simulink model "Gen3_J2_PMSM_Actuator"  (R2026b)
settings: Solver=ode23t  StopTime=1  MaxStep=1e-4  RelTol=1e-6  AbsTol=1e-8
model workspace (MAT data in the model file):
  p.Rs = 0.013
  p.Ld = 0.00019
  p.Lq = 0.00025
  p.pp = 6
  p.psi = 0.03
  p.Kt = 0.27
  p.N = 2
  p.Jtotal_motor = 0.0125
  p.Jm = 0.01
  p.Jload_test = 0.01
  p.Bm = 0
  p.Kpd = 0.19
  p.Kpq = 0.25
  p.Kid = 13
  p.Kiq = 13
  p.Imax = 1
  p.Vqmax = 1
  p.s = 1
  p.Kaw = 52
settings Model: Creator=rninh  LastModifiedBy=rninh

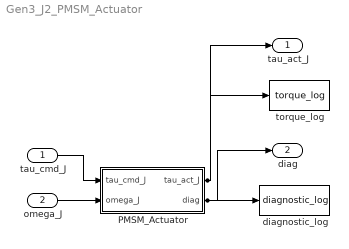
== system Gen3_J2_PMSM_Actuator ==
  tau_cmd_J : Inport  Unit=N*m  PortDimensions=1  Interpolate=off
  omega_J : Inport  Port=2  Unit=rad/s  PortDimensions=1  Interpolate=off
  PMSM_Actuator : Subsystem
  diagnostic_log : ToWorkspace  VariableName=diagnostic_log  SaveFormat=Timeseries  SampleTime=-1
  torque_log : ToWorkspace  VariableName=torque_log  SaveFormat=Timeseries  SampleTime=-1
  tau_act_J : Outport  Unit=N*m
  diag : Outport  Port=2
  wires:
  tau_cmd_J/1 -> PMSM_Actuator/1(tau_cmd_J)
  omega_J/1 -> PMSM_Actuator/2(omega_J)
  PMSM_Actuator/1(tau_act_J) -> tau_act_J/1, torque_log/1
  PMSM_Actuator/2(diag) -> diag/1, diagnostic_log/1

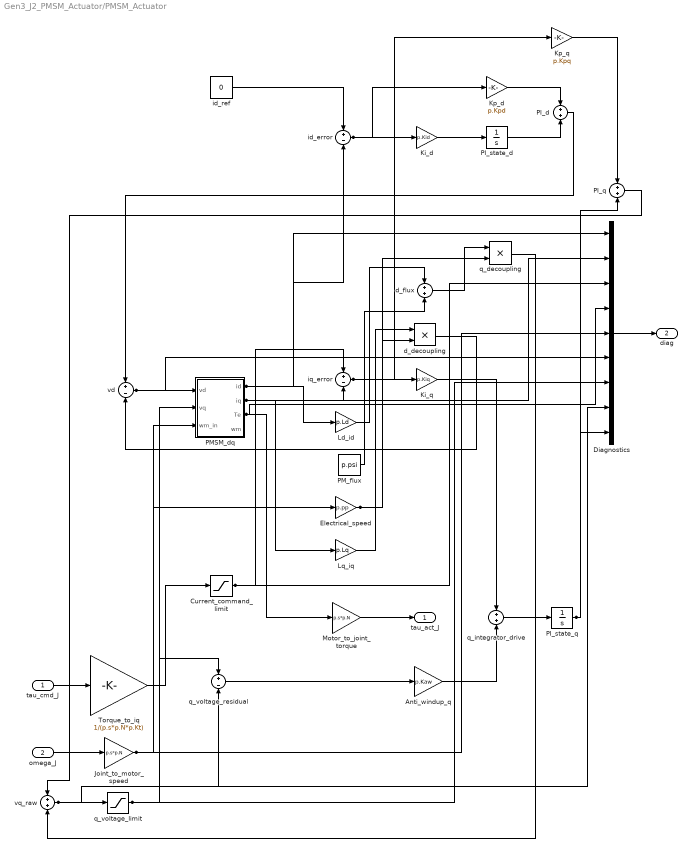
== system Gen3_J2_PMSM_Actuator/PMSM_Actuator ==
  tau_cmd_J : Inport  Unit=N*m  PortDimensions=1
  omega_J : Inport  Port=2  Unit=rad/s  PortDimensions=1
  Anti_windup_q : Gain  Gain=p.Kaw
  Current_command_limit : Saturate  UpperLimit=p.Imax  LowerLimit=-p.Imax
  Diagnostics : Mux  Inputs=9
  Electrical_speed : Gain  Gain=p.pp
  Joint_to_motor_speed : Gain  Gain=p.s*p.N
  Ki_d : Gain  Gain=p.Kid
  Ki_q : Gain  Gain=p.Kiq
  Kp_d : Gain  Gain=p.Kpd
  Kp_q : Gain  Gain=p.Kpq
  Ld_id : Gain  Gain=p.Ld
  Lq_iq : Gain  Gain=p.Lq
  Motor_to_joint_torque : Gain  Gain=p.s*p.N
  PI_d : Sum
  PI_q : Sum
  PI_state_d : Integrator
  PI_state_q : Integrator
  PMSM_dq : Subsystem
  PM_flux : Constant  Value=p.psi
  Torque_to_iq : Gain  Gain=1/(p.s*p.N*p.Kt)
  d_decoupling : Product
  d_flux : Sum
  id_error : Sum  Inputs=+-
  id_ref : Constant  Value=0
  iq_error : Sum  Inputs=+-
  q_decoupling : Product
  q_integrator_drive : Sum
  q_voltage_limit : Saturate  UpperLimit=p.Vqmax  LowerLimit=-p.Vqmax
  q_voltage_residual : Sum  Inputs=+-
  vd : Sum  Inputs=+-
  vq_raw : Sum
  tau_act_J : Outport  Unit=N*m  PortDimensions=1
  diag : Outport  Port=2
  wires:
  Joint_to_motor_speed/1 -> Electrical_speed/1, Diagnostics/5, PMSM_dq/3(wm_in)
  vd/1 -> Diagnostics/6, PMSM_dq/1(vd)
  PI_state_q/1 -> PI_q/2, Diagnostics/9
  tau_cmd_J/1 -> Torque_to_iq/1
  omega_J/1 -> Joint_to_motor_speed/1
  vq_raw/1 -> Diagnostics/8, q_voltage_residual/2, q_voltage_limit/1
  id_ref/1 -> id_error/1
  q_voltage_limit/1 -> q_voltage_residual/1, PMSM_dq/2(vq), Diagnostics/7
  Torque_to_iq/1 -> Current_command_limit/1
  d_flux/1 -> q_decoupling/1
  PMSM_dq/1(id) -> Diagnostics/1, id_error/2, Ld_id/1
  PMSM_dq/3(Te) -> Diagnostics/4, Motor_to_joint_torque/1
  PMSM_dq/2(iq) -> iq_error/2, Diagnostics/2, Lq_iq/1
  Current_command_limit/1 -> iq_error/1, Diagnostics/3
  q_voltage_residual/1 -> Anti_windup_q/1
  id_error/1 -> Kp_d/1, Ki_d/1
  iq_error/1 -> Kp_q/1, Ki_q/1
  Ld_id/1 -> d_flux/1
  PM_flux/1 -> d_flux/2
  Electrical_speed/1 -> q_decoupling/2, d_decoupling/2
  Lq_iq/1 -> d_decoupling/1
  Motor_to_joint_torque/1 -> tau_act_J/1
  Ki_d/1 -> PI_state_d/1
  d_decoupling/1 -> vd/2
  Ki_q/1 -> q_integrator_drive/1
  Anti_windup_q/1 -> q_integrator_drive/2
  Kp_d/1 -> PI_d/1
  PI_state_d/1 -> PI_d/2
  q_decoupling/1 -> vq_raw/2
  q_integrator_drive/1 -> PI_state_q/1
  Kp_q/1 -> PI_q/1
  PI_d/1 -> vd/1
  PI_q/1 -> vq_raw/1
  Diagnostics/1 -> diag/1

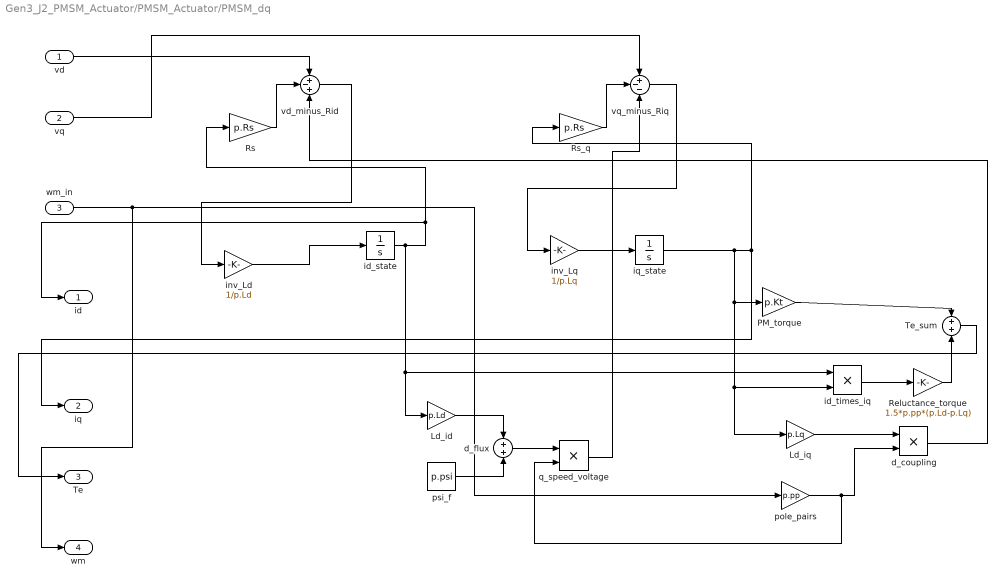
== system Gen3_J2_PMSM_Actuator/PMSM_Actuator/PMSM_dq ==
  vd : Inport
  vq : Inport  Port=2
  wm_in : Inport  Port=3
  Ld_id : Gain  Gain=p.Ld
  Ld_iq : Gain  Gain=p.Lq
  PM_torque : Gain  Gain=p.Kt
  Reluctance_torque : Gain  Gain=1.5*p.pp*(p.Ld-p.Lq)
  Rs : Gain  Gain=p.Rs
  Rs_q : Gain  Gain=p.Rs
  Te_sum : Sum
  d_coupling : Product
  d_flux : Sum
  id_state : Integrator
  id_times_iq : Product
  inv_Ld : Gain  Gain=1/p.Ld
  inv_Lq : Gain  Gain=1/p.Lq
  iq_state : Integrator
  pole_pairs : Gain  Gain=p.pp
  psi_f : Constant  Value=p.psi
  q_speed_voltage : Product
  vd_minus_Rid : Sum  Inputs=+-+
  vq_minus_Riq : Sum  Inputs=+--
  id : Outport
  iq : Outport  Port=2
  Te : Outport  Port=3
  wm : Outport  Port=4
  wires:
  wm_in/1 -> pole_pairs/1, wm/1
  vq/1 -> vq_minus_Riq/1
  vd/1 -> vd_minus_Rid/1
  psi_f/1 -> d_flux/2
  q_speed_voltage/1 -> vq_minus_Riq/3
  d_coupling/1 -> vd_minus_Rid/3
  Ld_iq/1 -> d_coupling/1
  Ld_id/1 -> d_flux/1
  Reluctance_torque/1 -> Te_sum/2
  Te_sum/1 -> Te/1
  d_flux/1 -> q_speed_voltage/1
  id_times_iq/1 -> Reluctance_torque/1
  inv_Ld/1 -> id_state/1
  inv_Lq/1 -> iq_state/1
  PM_torque/1 -> Te_sum/1
  pole_pairs/1 -> d_coupling/2, q_speed_voltage/2
  Rs/1 -> vd_minus_Rid/2
  Rs_q/1 -> vq_minus_Riq/2
  id_state/1 -> Rs/1, id/1, id_times_iq/1, Ld_id/1
  iq_state/1 -> Rs_q/1, iq/1, PM_torque/1, id_times_iq/2, Ld_iq/1
  vq_minus_Riq/1 -> inv_Lq/1
  vd_minus_Rid/1 -> inv_Ld/1
